simulink model "GFMUPS100k_CPP"  (R2024b)
settings: Solver=ode2  StartTime=0.0  StopTime=6  FixedStep=5e-7  RelTol=1e-3
model workspace (MAT data in the model file):
  amp = 0
  f1 = 1000
undefined symbols (not defined in the file or in its folder): DiscIntNeverNeededParam, L
libraries: spsIGBTDiodeLib x12, slpidlib x12, spsabctodq0Lib x10, spsSeriesRLCBranchLib x9, spsPLL3phLib x8, spsThreePhaseSeriesRLCBranchLib x8, spsDiodeLib x6, dspstat3 x5, spsVoltageMeasurementLib x4, spsThreePhaseVIMeasurementLib x4, spsPower3phInstantaneousLib x3, spsControlledCurrentSourceLib x3
(part 1 of 4)
settings Model: SimulationMode=accelerator  PacingRate=1000  Creator=Administrator  LastModifiedBy=zzc

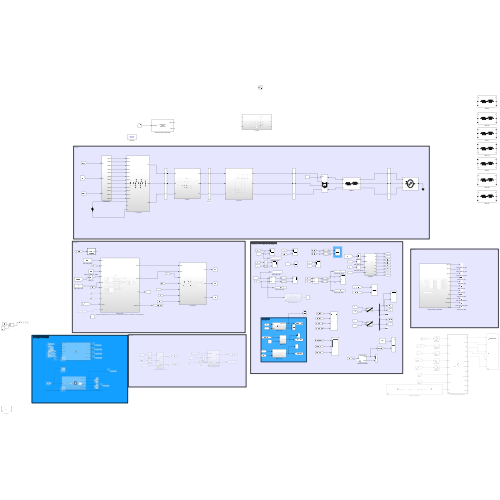
[thumbnail: Simulink's stored preview of the top-level diagram]
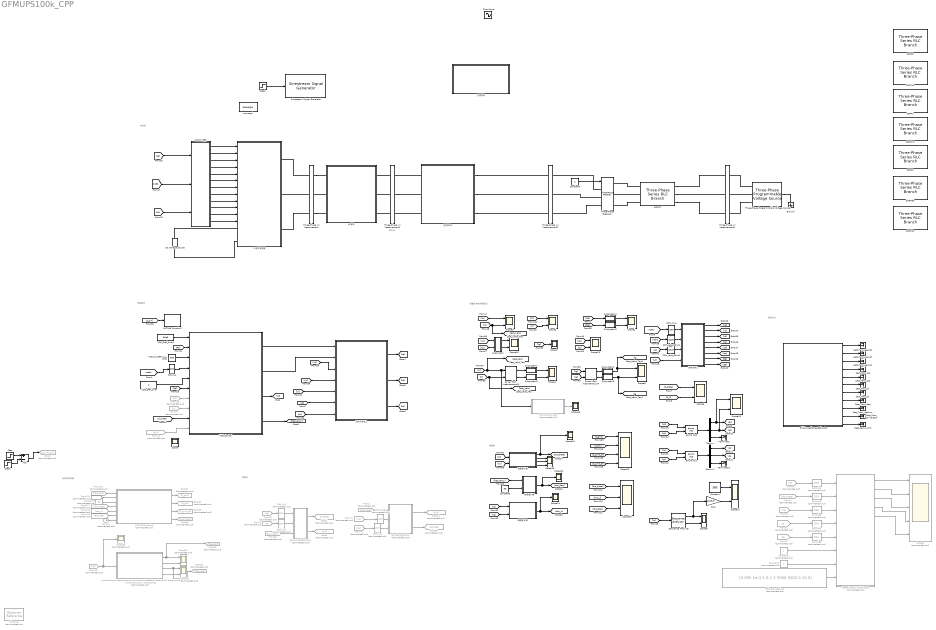
== system GFMUPS100k_CPP ==
  note: 阻抗估计
  note: PCC点
  note: 控制部分
  note: 主电路
  note: 相角差
  note: 测量与坐标转换部分
  note: 合闸信号判断
  note: 预同步
  A practical and fast sequence components detection scheme for three-phase unbalanced grid voltage.2021 : Subsystem  Commented=on
  Add : Sum  Inputs=+-
  Clock2 : Clock  Commented=on
  Constant : Constant  Value=380
  Constant1 : Constant  Commented=on
  Constant2 : Constant  Commented=on  Value=0
  Constant3 : Constant  Value=50
  Constant4 : Constant
  Constant5 : Constant  Commented=on  Value=50
  DC Voltage Source : spsDCVoltageSourceLib/DC Voltage Source  Amplitude=1500  Measurements=None
  Demux : Demux  Outputs=3
  Demux1 : Demux  Outputs=3
  Estimator_Settings : Constant  Commented=on  Value=[0.005 1e-4 5 0.1 5 5000 5000 0.15 0]
  From{10,40,74,121} (4 alike) : From  Commented=on  GotoTag=Vg  TagVisibility=global
  From11 : From  Commented=on  GotoTag=Qg  TagVisibility=global
  From116 : From  Commented=on  GotoTag=cha_freq
  From117 : From  Commented=on  GotoTag=cha_theta
  From118 : From  Commented=on  GotoTag=cha_U
  From119 : From  Commented=on  GotoTag=Mag_pos
  From12 : From  Commented=on  GotoTag=Pg  TagVisibility=global
  From120 : From  Commented=on  GotoTag=Mag_neg
  From2 : From  Commented=on  GotoTag=S_sync_en
  From26 : From  Commented=on  GotoTag=id
  From27 : From  Commented=on  GotoTag=iq
  From39 : From  Commented=on  GotoTag=S_sync_en
  From42 : From  Commented=on  GotoTag=Vs  TagVisibility=global
  From44 : From  Commented=on  GotoTag=d_U
  From73 : From  Commented=on  GotoTag=Vs  TagVisibility=global
  From8 : From  Commented=on  GotoTag=Vs  TagVisibility=global
  From9 : From  Commented=on  GotoTag=cha_theta
  Gain : Gain  Gain=sqrt(3/2)
  Goto39 : Goto  Commented=on  GotoTag=d_theta
  Goto40 : Goto  Commented=on  GotoTag=d_U
  Goto54 : Goto  Commented=on  GotoTag=Mag_pos
  Goto55 : Goto  Commented=on  GotoTag=Mag_neg
  Goto57 : Goto  Commented=on  GotoTag=S_grid
  Goto58 : Goto  Commented=on  GotoTag=S_sync_en
  Goto59 : Goto  Commented=on  GotoTag=S_sync_ok
  Goto60 : Goto  Commented=on  GotoTag=S_brk
  Goto7 : Goto  Commented=on  GotoTag=d_theta
  Goto8 : Goto  Commented=on  GotoTag=d_U
  Goto9 : Goto  Commented=on  GotoTag=S_sync_en
  Grid_Impedance_Estimator : Subsystem
  Ground : spsGroundLib/Ground  LConnTagsString=a
  IEC 62040-3-Test : Subsystem  Commented=on
  LC滤波 : Subsystem
  MATLAB Function2 : MATLAB Function  TreatAsAtomicUnit=on
  MATLAB Function3 : MATLAB Function  Commented=on  TreatAsAtomicUnit=on  SystemSampleTime=5e-05
  Observer : ObserverReference  Commented=on  ObserverModelName=GFMUPS100k_T1_Observer1
  Operating_Point_Estimator : MATLAB Function  Commented=on  TreatAsAtomicUnit=on
  "Power (3ph, Instantaneous)3" : spsPower3phInstantaneousLib/Power (3ph, Instantaneous)
  "Power (3ph, Instantaneous)4" : spsPower3phInstantaneousLib/Power (3ph, Instantaneous)
  SCR=1 : spsThreePhaseSeriesRLCBranchLib/Three-Phase Series RLC Branch  LConnTagsString=A|B|C  RConnTagsString=A|B|C  BranchType=RL  Resistance=0.1436835  Inductance=0.004573584  Capacitance=1e-6  Measurements=None
  SCR=1.5 : spsThreePhaseSeriesRLCBranchLib/Three-Phase Series RLC Branch  LConnTagsString=A|B|C  RConnTagsString=A|B|C  BranchType=RL  Resistance=0.095789  Inductance=0.003049056  Capacitance=1e-6  Measurements=None
  SCR=10 : spsThreePhaseSeriesRLCBranchLib/Three-Phase Series RLC Branch  LConnTagsString=A|B|C  RConnTagsString=A|B|C  BranchType=RL  Resistance=0.014368  Inductance=0.000457358  Capacitance=1e-6  Measurements=None
  SCR=2 : spsThreePhaseSeriesRLCBranchLib/Three-Phase Series RLC Branch  LConnTagsString=A|B|C  RConnTagsString=A|B|C  BranchType=RL  Resistance=0.047894  Inductance=0.001524528  Capacitance=1e-6  Measurements=None
  SCR=3 : spsThreePhaseSeriesRLCBranchLib/Three-Phase Series RLC Branch  LConnTagsString=A|B|C  RConnTagsString=A|B|C  BranchType=RL  Resistance=0.047894  Inductance=0.001524528  Capacitance=1e-6  Measurements=None
  SCR=30 : spsThreePhaseSeriesRLCBranchLib/Three-Phase Series RLC Branch  LConnTagsString=A|B|C  RConnTagsString=A|B|C  BranchType=RL  Resistance=0.004789  Inductance=0.000152453  Capacitance=1e-6  Measurements=None
  SCR=40 : spsThreePhaseSeriesRLCBranchLib/Three-Phase Series RLC Branch  LConnTagsString=A|B|C  RConnTagsString=A|B|C  BranchType=RL  Resistance=0.003592088  Inductance=0.0001143396  Capacitance=1e-6  Measurements=None
  SCR=5 : spsThreePhaseSeriesRLCBranchLib/Three-Phase Series RLC Branch  LConnTagsString=A|B|C  RConnTagsString=A|B|C  BranchType=RL  Resistance=0.028736674  Inductance=0.914716745e-3  Capacitance=1e-6  Measurements=None
  SVPWM调制 : Subsystem
  Sample{1..5} (5 alike) : ZeroOrderHold  Commented=on  SampleTime=1e-4
  Scope{,7,14,16,19..20} (6 alike) : Scope
  Scope{1..6,9..10,13,15,17} (11 alike) : Scope  NumInputPorts=2
  Scope11 : Scope  Commented=on  NumInputPorts=2
  Scope12 : Scope  Commented=on  NumInputPorts=2
  Scope18 : Scope  NumInputPorts=3
  Scope23 : Scope  Commented=on
  Scope24 : Scope  NumInputPorts=4
  Scope25 : Scope  NumInputPorts=3
  Scope8 : Scope  Commented=on  NumInputPorts=5
  Sequence Analyzer : eeSequenceAnalyzer/Sequence Analyzer  VariantControl=Variant1  LabelModeActiveChoice=Continuous  F=50  K=1  Seq=Positive  Ts=0
      settings: LibrarySourceBlock=ee_sl_lib/Measurements/Sequence Analyzer
  Sine Wave : Sin  SampleTime=0
  Sinestream Signal Generator : slctrl_signal/Sinestream Signal Generator  DiscreteTs=1e-4  BlockDataType=double  SignalSource=Block parameters  Frequencies=[20 40 60 100]  FreqUnits=Hz  Amplitudes=[1.07 1.07 1.07 1.07]  NumOfFreq=3  NumOfSignalPeriod=6  SinestreamType=sine  PhaseShift=0  PhaseShiftUnits=deg  ThreePhaseSignal=on  OutputFreqIndex=on  UseExternalTs=off  CompiledTsChoice=InternalTs  SinestreamSignalChoice=VariantSin3Phase
      settings: LibrarySourceBlock=slctrlblks/Signal Generation/Sinestream Signal Generator
  Step : Step  Time=0.3  SampleTime=0
  Step1 : Step  Time=0.85  SampleTime=0
  Step2 : Step  Time=0.5  SampleTime=0
  Subsystem : Subsystem
  Subsystem1 : Subsystem
  Subsystem2 : Subsystem
  Subsystem3 : Subsystem
  Subsystem4 : Subsystem
  Subsystem7 : Subsystem
  Subsystem8 : Subsystem
  Terminator : Terminator
  Terminator1 : Terminator
  Three-Phase Programmable Voltage Source : spsThreePhaseProgrammableVoltageSourceLib/Three-Phase Programmable Voltage Source  PositiveSequence="[380  0 50]"  VariationEntity=None  VariationType=Step  VariationTypeAlt=Step  VariationStep=-0.2  VariationRate=10  VariationMagnitude=0.3  VariationFrequency=2  VariationTiming=[1.5 2.4]  VariationPhaseA=off  Amplitudes=[1 0.8 1.2 1.0]  TimeValues=[0 0.1 0.15 0.2]  HarmonicGeneration=off  HarmonicA=[3 0.2 -25 0]  HarmonicB=[2 0.15 35 2]  Timing="[0.05  3]"  BusType=swing  Pref=0  Qref=0  Qmin=-inf  Qmax=inf
  Three-Phase V-I Measurement : spsThreePhaseVIMeasurementLib/Three-Phase V-I Measurement  VoltageMeasurement=no  SetLabelV=off  LabelV=Vabc  Vpu=off  VpuLL=off  CurrentMeasurement=yes  SetLabelI=on  LabelI=Iabc  Ipu=off  Pbase=100e6  Vbase=500e3  OutputType=Complex  PhasorSimulation=off  PSBequivalent=0
  Three-Phase V-I Measurement1 : spsThreePhaseVIMeasurementLib/Three-Phase V-I Measurement  VoltageMeasurement=phase-to-ground  SetLabelV=on  LabelV=Vs  Vpu=off  VpuLL=off  CurrentMeasurement=yes  SetLabelI=on  LabelI=Is  Ipu=off  Pbase=100e6  Vbase=500e3  OutputType=Complex  PhasorSimulation=off  PSBequivalent=0
  Three-Phase V-I Measurement2 : spsThreePhaseVIMeasurementLib/Three-Phase V-I Measurement  VoltageMeasurement=phase-to-ground  SetLabelV=on  LabelV=Vg  Vpu=off  VpuLL=off  CurrentMeasurement=yes  SetLabelI=on  LabelI=Ig  Ipu=off  Pbase=100e6  Vbase=500e3  OutputType=Complex  PhasorSimulation=off  PSBequivalent=0
  Three-Phase V-I Measurement4 : spsThreePhaseVIMeasurementLib/Three-Phase V-I Measurement  VoltageMeasurement=phase-to-ground  SetLabelV=on  LabelV=V1  Vpu=off  VpuLL=off  CurrentMeasurement=yes  SetLabelI=on  LabelI=I1  Ipu=off  Pbase=100e6  Vbase=500e3  OutputType=Complex  PhasorSimulation=off  PSBequivalent=0
  Three-Phase Breaker1 : spsThreePhaseBreakerLib/Three-Phase Breaker  InitialState=closed  SwitchA=on  SwitchB=on  SwitchC=on  SwitchTimes="[1  2]"  External=on  BreakerResistance=1e-6  SnubberResistance=1e6  SnubberCapacitance=inf  Measurements=None
  VSG_Control : Subsystem
      settings: AttributesFormatString=Reviewed discrete VSG, Ts=100 us; Q-U retuned to 0.5 Hz for real NPC; L1/R1 bypassed
  VSG_Qref_0var : Constant  Value=0  SampleTime=100e-6
  VSG_Qref_0var1 : Constant  Value=80e3  SampleTime=100e-6
  VSG_Un_380V_LL_RMS : Constant  Value=380  SampleTime=100e-6
  ZOH_Iabc_50us1 : ZeroOrderHold  SampleTime=50e-6
  ZOH_Iabc_50us2 : ZeroOrderHold  SampleTime=50e-6
  ZOH_Vs : ZeroOrderHold  SampleTime=5e-05
  ZOH_Vs{1..4} (4 alike) : ZeroOrderHold  Commented=on  SampleTime=5e-05
  ZOH_Vs_1 : ZeroOrderHold  SampleTime=5e-6
  Zest_Term_Lg_hat : Terminator
  Zest_Term_Pg : Terminator
  Zest_Term_Qg : Terminator
  Zest_Term_Rg_hat : Terminator
  Zest_Term_Xg_hat : Terminator
  Zest_Term_converged : Terminator
  Zest_Term_detJ : Terminator
  Zest_Term_f1 : Terminator
  Zest_Term_f2 : Terminator
  Zest_Term_iterNum : Terminator
  Zest_Term_valid : Terminator
  abc to dq0 : spsabctodq0Lib/abc to dq0  Alignment=90 degrees behind phase A axis
  abc to dq1 : spsabctodq0Lib/abc to dq0  Alignment=90 degrees behind phase A axis
  powergui : spspowerguiLib/powergui  Priority=1  SimulationMode=Discrete  SampleTime=5e-7  frequency=60  Iterations=50  frequencyindice=0  Pbase=100e6  ErrMax=1e-4  UnitsV=kV  UnitsW=MW  buscounter=0  FunctionMessages=off  echomessages=off  EnableUseOfTLC=off  CurrentSourceSwitches=off  DisableSnubberDevices=off  DisableRonSwitches=off  DisableVfSwitches=off  DisplayEquations=off  AutomaticDiscreteSolvers=off  SolverType=Tustin/Backward Euler (TBE)  Interpol=off  ExternalGateDelay=off  methode=off  Ts=100  x0status=blocks  SPID=on  SwTol=0  HookPort=off  NonlinearTolerance=1e-4  nMaxIteration=100  ContinueOnMaxIteration=off  RestoreLinks=warning  ResistiveCurrentMeasurement=off  Frange=[0:2:500]  Ylog=off  Xlog=on  ShowGrid=off  save=off  variable=ZData  structure=0  ZoomFFT=off  StartTime=0.0  cycles=1  DisplayStyle=1  fundamental=60  FreqAxis=off  MaxFrequency=1000  frequencyindicesteady=1  RmsSteady=1  display=off
  三电平逆变器 : Subsystem
  双闭环控制1 : Subsystem
  坐标变换1 : Subsystem
  基于自适应虚拟电流 : Subsystem  Commented=on
  基于转dq的预同步控制1 : Subsystem  Commented=on
  幅值差计算 : Subsystem
  正序扰动 : Subsystem
  正序扰动1 : Subsystem
  相角差计算 : Subsystem
  频率差计算 : Subsystem
  tag scope: Pg=global, Qg=global, Vgd=global, Vgq=global, Vsd=global, Vsq=global, Zest_ILabc=global, Zest_Iuabc=global, Zest_Vabc=global
  wires:
  SVPWM调制/1(PWM1) -> 三电平逆变器/1(pwm1)
  SVPWM调制/2(PWM2) -> 三电平逆变器/2(pwm2)
  SVPWM调制/3(PWM3) -> 三电平逆变器/3(pwm3)
  SVPWM调制/4(PWM4) -> 三电平逆变器/4(pwm4)
  SVPWM调制/5(PWM5) -> 三电平逆变器/5(pwm5)
  SVPWM调制/6(PWM6) -> 三电平逆变器/6(pwm6)
  SVPWM调制/7(PWM7) -> 三电平逆变器/7(pwm7)
  SVPWM调制/8(PWM8) -> 三电平逆变器/8(pwm8)
  SVPWM调制/9(PWM9) -> 三电平逆变器/9(pwm9)
  SVPWM调制/10(PWM10) -> 三电平逆变器/10(pwm10)
  SVPWM调制/11(PWM11) -> 三电平逆变器/11(pwm11)
  SVPWM调制/12(PWM12) -> 三电平逆变器/12(pwm12)
  VSG_Un_380V_LL_RMS/1 -> VSG_Control/3(Un)
  VSG_Qref_0var/1 -> VSG_Control/5(Qref)
  VSG_Control/3(wt) -> [wt]
  坐标变换1/2(vq) -> [vq]
  坐标变换1/5(isd) -> [isd]
  坐标变换1/1(vd) -> [vd]
  坐标变换1/7(Pe) -> [Pe]
  坐标变换1/8(Qe) -> [Qe]
  [wt] -> 坐标变换1/4(wt)
  坐标变换1/4(iq) -> [iq]
  [Iabc] -> ZOH_Iabc_50us1/1
  [Is] -> ZOH_Iabc_50us2/1
  坐标变换1/6(isq) -> [isq]
  坐标变换1/3(id) -> [id]
  [Vcabc] -> ZOH_Vs_1/1
  ZOH_Vs_1/1 -> 坐标变换1/1(Vs)
  ZOH_Iabc_50us1/1 -> 坐标变换1/2(Iabc)
  ZOH_Iabc_50us2/1 -> 坐标变换1/3(Is)
  [Ua] -> SVPWM调制/1(ua)
  [Ub] -> SVPWM调制/2(ub)
  [Uc] -> SVPWM调制/3(uc)
  [Pe] -> VSG_Control/2(Pe)
  [Qe] -> VSG_Control/6(Qe)
  From26/1 -> VSG_Control/7(id)
  From27/1 -> VSG_Control/8(iq)
  [Vcabc] -> ZOH_Vs/1
  ZOH_Vs/1 -> VSG_Control/4(Vs)
  VSG_Control/4(frequency) -> [frequency]
  [iq] -> 双闭环控制1/6(iq)
  双闭环控制1/3(UC) -> [Uc]
  [id] -> 双闭环控制1/5(id)
  双闭环控制1/2(UB) -> [Ub]
  [vd] -> 双闭环控制1/3(Vd)
  双闭环控制1/1(UA) -> [Ua]
  [wt] -> 双闭环控制1/7(wt)
  [vq] -> 双闭环控制1/4(Vq)
  From40/1 -> ZOH_Vs1/1
  基于转dq的预同步控制1/1(c_theta) -> Goto7/1
  From42/1 -> ZOH_Vs2/1
  基于转dq的预同步控制1/2(d_U) -> Goto8/1
  From39/1 -> 基于转dq的预同步控制1/3(presignal)
  [d_theta] -> VSG_Control/9(d_theta)
  From44/1 -> VSG_Control/10(d_U)
  Add/1 -> Goto9/1
  Step/1 -> Add/1
  Step1/1 -> Add/2
  [S_sync_ok] -> Scope24/3
  "Power (3ph, Instantaneous)4"/1 -> Subsystem1/1(In1)
  [cha_freq] -> Scope25/3
  [V1] -> 相角差计算/2(abc1)
  [Vl] -> Scope2/1
  相角差计算/3(Out3) -> Scope18/2
  [Vl] -> IEC 62040-3-Test/1(In1), "Power (3ph, Instantaneous)3"/1, [Zest_Vabc]
  Subsystem/2(Out2) -> Scope10/2
  Subsystem/1(Out1) -> Scope10/1
  [Vs] -> Subsystem/1(In1)
  "Power (3ph, Instantaneous)3"/2 -> Subsystem8/1(In1)
  "Power (3ph, Instantaneous)4"/2 -> Subsystem2/1(In1)
  "Power (3ph, Instantaneous)3"/1 -> Subsystem7/1(In1)
  [Ig] -> "Power (3ph, Instantaneous)4"/2
  [Vg] -> Scope13/1
  [frequency] -> 频率差计算/1(In1)
  [Vg] -> Subsystem/2(In2)
  频率差计算/1(Out1) -> Scope20/1, [cha_freq]
  [Vs] -> 相角差计算/1(abc)
  相角差计算/1(dete_theta) -> Scope19/1, [cha_theta]
  [S_grid] -> Scope24/1
  相角差计算/4(Out4) -> Scope18/3
  [Vs] -> Scope3/1  "Vs"
  [Vg] -> 幅值差计算/2(In2)
  [S_sync_en] -> Scope24/4
  IEC 62040-3-Test/1(Out1) -> Scope16/1
  [Il] -> Scope2/2
  幅值差计算/1(Out1) -> Scope14/1, [cha_U]
  [Vg] -> Scope7/1
  [Il] -> "Power (3ph, Instantaneous)3"/2, [Zest_ILabc]
  [cha_theta] -> Scope25/1
  Constant3/1 -> 频率差计算/2(In2)
  相角差计算/2(Out2) -> Scope18/1
  [Ig] -> Scope13/2
  [Vg] -> "Power (3ph, Instantaneous)4"/1
  [S_brk] -> Scope24/2
  [Vs] -> 幅值差计算/1(In1)
  [cha_U] -> Scope25/2
  Subsystem1/1(Out1) -> [Pg], Scope5/1  "Pg"
  Subsystem2/1(Out1) -> [Qg], Scope5/2  "Qg"
  Subsystem7/1(Out1) -> Scope4/1
  Subsystem8/1(Out1) -> Scope4/2
  [Pe] -> Subsystem4/1(In1)  "Pe"
  [Qe] -> Subsystem3/1(In1)  "Qe"
  ZOH_Vs1/1 -> 基于转dq的预同步控制1/1(Vg)
  ZOH_Vs2/1 -> 基于转dq的预同步控制1/2(Vabc)
  [Is] -> Scope3/2, [Zest_Iuabc]  "Is"
  VSG_Control/1(Vdref) -> 双闭环控制1/1(Vdref)
  VSG_Control/2(Vqref) -> 双闭环控制1/2(Vqref)
  MATLAB Function3/4(S_sync_en) -> Goto58/1
  From120/1 -> MATLAB Function3/2(v2_pu)
  A practical and fast sequence components detection scheme for three-phase unbalanced grid voltage.2021/4(Angle_neg) -> Scope12/2
  MATLAB Function3/2(S_brk) -> Goto60/1
  Constant5/1 -> MATLAB Function3/3(freq_hz)
  Clock2/1 -> MATLAB Function3/7(t)
  From116/1 -> MATLAB Function3/6(d_f)
  MATLAB Function3/1(S_grid) -> Goto57/1
  A practical and fast sequence components detection scheme for three-phase unbalanced grid voltage.2021/2(Angle_pos) -> Scope11/2
  From121/1 -> Scope23/1, A practical and fast sequence components detection scheme for three-phase unbalanced grid voltage.2021/1(In1)
  A practical and fast sequence components detection scheme for three-phase unbalanced grid voltage.2021/3(Mag_neg) -> Scope12/1, Goto55/1
  A practical and fast sequence components detection scheme for three-phase unbalanced grid voltage.2021/1(Mag_pos) -> Scope11/1, Goto54/1
  From117/1 -> MATLAB Function3/4(d_theta)
  From118/1 -> MATLAB Function3/5(d_U)
  From119/1 -> MATLAB Function3/1(v1_pu)
  MATLAB Function3/3(S_sync_ok) -> Goto59/1
  From2/1 -> 基于自适应虚拟电流/1(presignal)
  From74/1 -> ZOH_Vs4/1
  基于自适应虚拟电流/2(deta_w) -> Goto39/1
  基于自适应虚拟电流/1(deta_U) -> Goto40/1
  From73/1 -> ZOH_Vs3/1
  [d_theta] -> Scope6/1
  [d_U] -> Scope6/2
  ZOH_Vs3/1 -> 基于自适应虚拟电流/2(Vs_abc)
  ZOH_Vs4/1 -> 基于自适应虚拟电流/3(Vg_abc1)
  [S_brk] -> MATLAB Function2/1(S_brk)
  Step2/1 -> Sinestream Signal Generator/1
  Grid_Impedance_Estimator/1(Rg_hat) -> Zest_Term_Rg_hat/1
  Grid_Impedance_Estimator/2(Xg_hat) -> Zest_Term_Xg_hat/1
  Grid_Impedance_Estimator/3(Lg_hat) -> Zest_Term_Lg_hat/1
  Grid_Impedance_Estimator/4(Pg) -> Zest_Term_Pg/1
  Grid_Impedance_Estimator/5(Qg) -> Zest_Term_Qg/1
  Grid_Impedance_Estimator/6(f1) -> Zest_Term_f1/1
  Grid_Impedance_Estimator/7(f2) -> Zest_Term_f2/1
  Grid_Impedance_Estimator/8(detJ) -> Zest_Term_detJ/1
  Grid_Impedance_Estimator/9(iterNum) -> Zest_Term_iterNum/1
  Grid_Impedance_Estimator/10(converged) -> Zest_Term_converged/1
  Grid_Impedance_Estimator/11(valid) -> Zest_Term_valid/1
  From8/1 -> Sample1/1  "Vs"
  From9/1 -> Sample2/1
  From10/1 -> Sample3/1
  From11/1 -> Sample5/1
  From12/1 -> Sample4/1
  Constant2/1 -> Operating_Point_Estimator/7(reset)
  Sample1/1 -> Operating_Point_Estimator/1(E)
  Sample2/1 -> Operating_Point_Estimator/2(theta)
  Sample3/1 -> Operating_Point_Estimator/3(Vg)
  Sample4/1 -> Operating_Point_Estimator/4(Pg)
  Sample5/1 -> Operating_Point_Estimator/5(Qg)
  Constant1/1 -> Operating_Point_Estimator/6(enable)
  Estimator_Settings/1 -> Operating_Point_Estimator/8(cfg)
  Operating_Point_Estimator/1(E0) -> Scope8/1
  Operating_Point_Estimator/2(theta0) -> Scope8/2
  Operating_Point_Estimator/3(Vg0) -> Scope8/3
  Operating_Point_Estimator/4(Pg0) -> Scope8/4
  Operating_Point_Estimator/5(Qg0) -> Scope8/5
  Constant4/1 -> Three-Phase Breaker1/1
  [V1] -> abc to dq0/1
  [wt] -> abc to dq0/2
  Demux/2 -> Scope15/2, [Vgq]
  abc to dq0/1 -> Demux/1
  Demux/3 -> Terminator/1
  Demux/1 -> Scope15/1, [Vgd]
  Demux1/3 -> Terminator1/1
  abc to dq1/1 -> Demux1/1
  Demux1/2 -> [Vsq]
  [wt] -> abc to dq1/2
  [Vs] -> abc to dq1/1
  Demux1/1 -> [Vsd]
  Constant/1 -> Scope17/1
  Gain/1 -> Scope17/2
  Sequence Analyzer/2 -> Scope9/2
  [Vs] -> Sequence Analyzer/1  "Vs"
  Sequence Analyzer/1 -> Gain/1, Scope9/1
  VSG_Qref_0var1/1 -> VSG_Control/1(Pref)
  Subsystem4/1(Out1) -> Scope1/1  "Pg"
  Subsystem3/1(Out1) -> Scope1/2  "Qg"
  connections:
  DC Voltage Source/RConn1 -- 三电平逆变器/LConn1
  DC Voltage Source/LConn1 -- 三电平逆变器/LConn3
  Three-Phase V-I Measurement/LConn1 -- 三电平逆变器/RConn1
  Three-Phase V-I Measurement/LConn2 -- 三电平逆变器/RConn2
  Three-Phase V-I Measurement/LConn3 -- 三电平逆变器/RConn3
  LC滤波/LConn2 -- Three-Phase V-I Measurement/RConn2
  Three-Phase V-I Measurement/RConn1 -- LC滤波/LConn1
  Three-Phase V-I Measurement/RConn3 -- LC滤波/LConn3
  Three-Phase V-I Measurement1/LConn1 -- LC滤波/RConn1
  Three-Phase V-I Measurement1/LConn2 -- LC滤波/RConn2
  Three-Phase V-I Measurement1/LConn3 -- LC滤波/RConn3
  Three-Phase Breaker1/LConn2 -- Three-Phase V-I Measurement2/RConn2
  Three-Phase Breaker1/LConn3 -- Three-Phase V-I Measurement2/RConn3
  SCR=2/RConn2 -- Three-Phase V-I Measurement4/LConn2
  Three-Phase Breaker1/LConn1 -- Three-Phase V-I Measurement2/RConn1
  Three-Phase Programmable Voltage Source/LConn1 -- Ground/LConn1
  正序扰动1/RConn3 -- Three-Phase V-I Measurement2/LConn3
  正序扰动1/LConn1 -- Three-Phase V-I Measurement1/RConn1
  Three-Phase V-I Measurement1/RConn2 -- 正序扰动1/LConn2
  正序扰动1/LConn3 -- Three-Phase V-I Measurement1/RConn3
  SCR=2/LConn1 -- Three-Phase Breaker1/RConn1
  SCR=2/LConn2 -- Three-Phase Breaker1/RConn2
  SCR=2/LConn3 -- Three-Phase Breaker1/RConn3
  Three-Phase Programmable Voltage Source/RConn1 -- Three-Phase V-I Measurement4/RConn1
  Three-Phase Programmable Voltage Source/RConn2 -- Three-Phase V-I Measurement4/RConn2
  Three-Phase Programmable Voltage Source/RConn3 -- Three-Phase V-I Measurement4/RConn3
  SCR=2/RConn3 -- Three-Phase V-I Measurement4/LConn3
  SCR=2/RConn1 -- Three-Phase V-I Measurement4/LConn1
  正序扰动1/RConn1 -- Three-Phase V-I Measurement2/LConn1
  正序扰动1/RConn2 -- Three-Phase V-I Measurement2/LConn2

== system GFMUPS100k_CPP/A practical and fast sequence components detection scheme for three-phase unbalanced grid voltage.2021 ==
  note: 滤波
  In1 : Inport
  MATLAB Function1 : MATLAB Function  TreatAsAtomicUnit=on
  Mux : Mux  Inputs=3
  PLL (3ph) : spsPLL3phLib/PLL (3ph)  Fmin=45  Par_Init=[0, 60]  ParK=[180, 3200, 1]  TcD=1e-4  MaxRateChangeFreq=12  FilterCutOffFreq=25  Ts=0  AGC=on
  Subsystem : Subsystem
  Subsystem1 : Subsystem
  T1\T2矩阵变换 : MATLAB Function  TreatAsAtomicUnit=on
  Terminator : Terminator
  Ubeta计算 : Subsystem
  标幺化1 : Subsystem
  Mag_pos : Outport
  Angle_pos : Outport  Port=2
  Mag_neg : Outport  Port=3
  Angle_neg : Outport  Port=4
  wires:
  Mux/1 -> T1\T2矩阵变换/2(U_beta)
  Ubeta计算/1(uA_beta) -> Mux/1
  Ubeta计算/3(uC_beta) -> Mux/3
  标幺化1/1(U_alpha) -> Ubeta计算/1(In1), T1\T2矩阵变换/1(U_alpha)
  Ubeta计算/2(uB_beta) -> Mux/2
  In1/1 -> 标幺化1/1(In1)
  T1\T2矩阵变换/1(U_pos) -> PLL (3ph)/1, Subsystem/1(abc)
  PLL (3ph)/1 -> Terminator/1
  MATLAB Function1/1(Mag_pos) -> Mag_pos/1
  MATLAB Function1/2(Angle_pos) -> Angle_pos/1
  MATLAB Function1/3(Mag_neg) -> Mag_neg/1
  MATLAB Function1/4(Angle_neg) -> Angle_neg/1
  Subsystem1/2(uq_fliter) -> MATLAB Function1/4(Uq_neg)
  T1\T2矩阵变换/2(U_neg) -> Subsystem1/1(abc)
  Subsystem1/1(ud_fliter) -> MATLAB Function1/3(Ud_neg)
  Subsystem/2(uq_fliter) -> MATLAB Function1/2(Uq_pos)
  PLL (3ph)/2 -> Subsystem1/2(In1), MATLAB Function1/5(wt)
  Subsystem/1(ud_fliter) -> MATLAB Function1/1(Ud_pos)

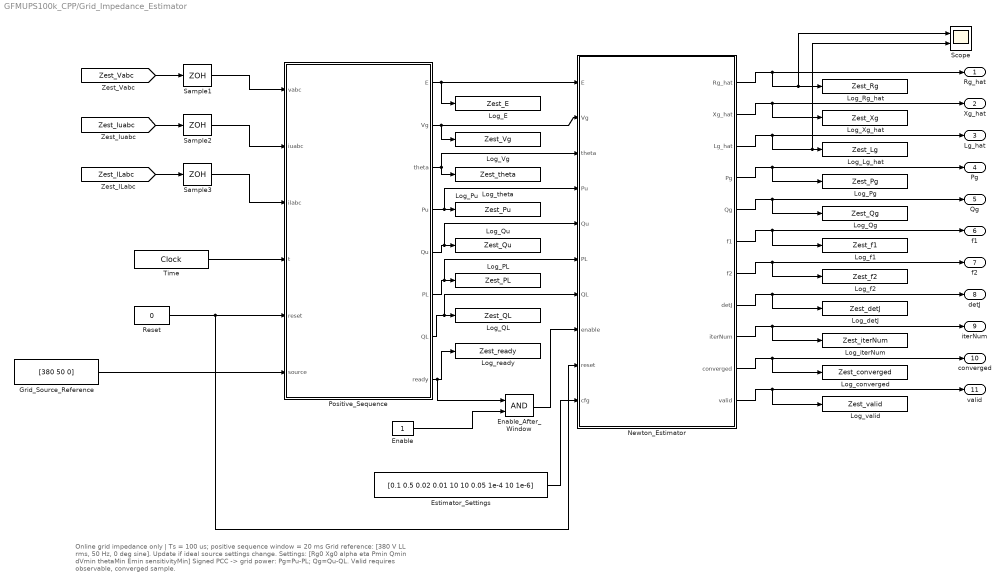
== system GFMUPS100k_CPP/Grid_Impedance_Estimator ==
  note: Online grid impedance only | Ts = 100 us; positive sequence window = 20 ms
      | Grid reference: [380 V LL rms, 50 Hz, 0 deg sine]. Update if ideal source settings change.
      | Settings: [Rg0 Xg0 alpha eta Pmin Qmin dVmin thetaMin Emin sensitivityMin]
      | Signed PCC -> grid power: Pg=Pu-PL; Qg=Qu-QL. Valid requires observable, converged sample.
  Enable : Constant  OutDataTypeStr=boolean
  Enable_After_Window : Logic
  Estimator_Settings : Constant  Value=[0.1 0.5 0.02 0.01 10 10 0.05 1e-4 10 1e-6]
  Grid_Source_Reference : Constant  Value=[380 50 0]
  Log_E : ToWorkspace  VariableName=Zest_E  SaveFormat=Timeseries  SampleTime=-1
  Log_Lg_hat : ToWorkspace  VariableName=Zest_Lg  SaveFormat=Timeseries  SampleTime=-1
  Log_PL : ToWorkspace  VariableName=Zest_PL  SaveFormat=Timeseries  SampleTime=-1
  Log_Pg : ToWorkspace  VariableName=Zest_Pg  SaveFormat=Timeseries  SampleTime=-1
  Log_Pu : ToWorkspace  VariableName=Zest_Pu  SaveFormat=Timeseries  SampleTime=-1
  Log_QL : ToWorkspace  VariableName=Zest_QL  SaveFormat=Timeseries  SampleTime=-1
  Log_Qg : ToWorkspace  VariableName=Zest_Qg  SaveFormat=Timeseries  SampleTime=-1
  Log_Qu : ToWorkspace  VariableName=Zest_Qu  SaveFormat=Timeseries  SampleTime=-1
  Log_Rg_hat : ToWorkspace  VariableName=Zest_Rg  SaveFormat=Timeseries  SampleTime=-1
  Log_Vg : ToWorkspace  VariableName=Zest_Vg  SaveFormat=Timeseries  SampleTime=-1
  Log_Xg_hat : ToWorkspace  VariableName=Zest_Xg  SaveFormat=Timeseries  SampleTime=-1
  Log_converged : ToWorkspace  VariableName=Zest_converged  SaveFormat=Timeseries  SampleTime=-1
  Log_detJ : ToWorkspace  VariableName=Zest_detJ  SaveFormat=Timeseries  SampleTime=-1
  Log_f1 : ToWorkspace  VariableName=Zest_f1  SaveFormat=Timeseries  SampleTime=-1
  Log_f2 : ToWorkspace  VariableName=Zest_f2  SaveFormat=Timeseries  SampleTime=-1
  Log_iterNum : ToWorkspace  VariableName=Zest_iterNum  SaveFormat=Timeseries  SampleTime=-1
  Log_ready : ToWorkspace  VariableName=Zest_ready  SaveFormat=Timeseries  SampleTime=-1
  Log_theta : ToWorkspace  VariableName=Zest_theta  SaveFormat=Timeseries  SampleTime=-1
  Log_valid : ToWorkspace  VariableName=Zest_valid  SaveFormat=Timeseries  SampleTime=-1
  Newton_Estimator : MATLAB Function  TreatAsAtomicUnit=on
  Positive_Sequence : MATLAB Function  TreatAsAtomicUnit=on
  Reset : Constant  Value=0
  Sample1 : ZeroOrderHold  SampleTime=1e-4
  Sample2 : ZeroOrderHold  SampleTime=1e-4
  Sample3 : ZeroOrderHold  SampleTime=1e-4
  Scope : Scope  NumInputPorts=2
  Time : DigitalClock  SampleTime=1e-4
  Rg_hat : Outport
  Xg_hat : Outport  Port=2
  Lg_hat : Outport  Port=3
  Pg : Outport  Port=4
  Qg : Outport  Port=5
  f1 : Outport  Port=6
  f2 : Outport  Port=7
  detJ : Outport  Port=8
  iterNum : Outport  Port=9
  converged : Outport  Port=10
  valid : Outport  Port=11
  wires:
  [Zest_Vabc] -> Sample1/1
  [Zest_Iuabc] -> Sample2/1
  [Zest_ILabc] -> Sample3/1
  Sample1/1 -> Positive_Sequence/1(vabc)
  Sample2/1 -> Positive_Sequence/2(iuabc)
  Sample3/1 -> Positive_Sequence/3(ilabc)
  Time/1 -> Positive_Sequence/4(t)
  Reset/1 -> Positive_Sequence/5(reset), Newton_Estimator/9(reset)
  Grid_Source_Reference/1 -> Positive_Sequence/6(source)
  Positive_Sequence/1(E) -> Log_E/1, Newton_Estimator/1(E)
  Positive_Sequence/2(Vg) -> Newton_Estimator/2(Vg), Log_Vg/1
  Positive_Sequence/3(theta) -> Newton_Estimator/3(theta), Log_theta/1
  Positive_Sequence/4(Pu) -> Newton_Estimator/4(Pu), Log_Pu/1
  Positive_Sequence/5(Qu) -> Newton_Estimator/5(Qu), Log_Qu/1
  Positive_Sequence/6(PL) -> Newton_Estimator/6(PL), Log_PL/1
  Positive_Sequence/7(QL) -> Newton_Estimator/7(QL), Log_QL/1
  Positive_Sequence/8(ready) -> Log_ready/1, Enable_After_Window/1
  Enable/1 -> Enable_After_Window/2
  Enable_After_Window/1 -> Newton_Estimator/8(enable)
  Estimator_Settings/1 -> Newton_Estimator/10(cfg)
  Newton_Estimator/1(Rg_hat) -> Rg_hat/1, Scope/1, Log_Rg_hat/1
  Newton_Estimator/2(Xg_hat) -> Xg_hat/1, Log_Xg_hat/1
  Newton_Estimator/3(Lg_hat) -> Lg_hat/1, Scope/2, Log_Lg_hat/1
  Newton_Estimator/4(Pg) -> Pg/1, Log_Pg/1
  Newton_Estimator/5(Qg) -> Qg/1, Log_Qg/1
  Newton_Estimator/6(f1) -> f1/1, Log_f1/1
  Newton_Estimator/7(f2) -> f2/1, Log_f2/1
  Newton_Estimator/8(detJ) -> detJ/1, Log_detJ/1
  Newton_Estimator/9(iterNum) -> iterNum/1, Log_iterNum/1
  Newton_Estimator/10(converged) -> converged/1, Log_converged/1
  Newton_Estimator/11(valid) -> valid/1, Log_valid/1

== system GFMUPS100k_CPP/IEC 62040-3-Test ==
  In1 : Inport
  Add1 : Sum
  Demux : Demux  Outputs=3
  Gain : Gain  Gain=1/563
  PLL (3ph) : spsPLL3phLib/PLL (3ph)  Fmin=45  Par_Init=[0, 60]  ParK=[180, 3200, 1]  TcD=1e-4  MaxRateChangeFreq=12  FilterCutOffFreq=25  Ts=0  AGC=on
  Scope : Scope
  Sqrt : Sqrt
  Terminator : Terminator
  Terminator1 : Terminator
  abc to dq0 : spsabctodq0Lib/abc to dq0  Alignment=90 degrees behind phase A axis
  Out1 : Outport
  wires:
  Gain/1 -> abc to dq0/1, Scope/1
  Add1/1 -> Sqrt/1
  Demux/2 -> Add1/2
  In1/1 -> PLL (3ph)/1, Gain/1
  Demux/1 -> Add1/1
  Demux/3 -> Terminator/1
  abc to dq0/1 -> Demux/1
  Sqrt/1 -> Out1/1
  PLL (3ph)/2 -> abc to dq0/2
  PLL (3ph)/1 -> Terminator1/1

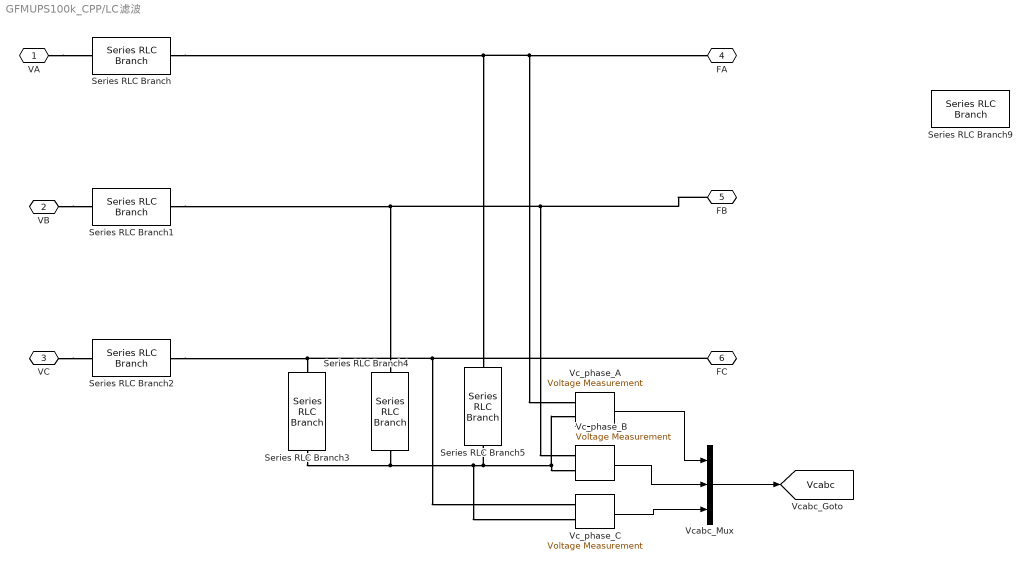
== system GFMUPS100k_CPP/LC滤波 ==
  Series RLC Branch : spsSeriesRLCBranchLib/Series RLC Branch  LConnTagsString=__new0  RConnTagsString=__new0  BranchType=RL  Resistance=0.01  Inductance=182e-6  SetiL0=off  InitialCurrent=0  Capacitance=1e-6  Setx0=off  InitialVoltage=0  Measurements=None
  Series RLC Branch1 : spsSeriesRLCBranchLib/Series RLC Branch  LConnTagsString=__new0  RConnTagsString=__new0  BranchType=RL  Resistance=0.01  Inductance=182e-6  SetiL0=off  InitialCurrent=0  Capacitance=1e-6  Setx0=off  InitialVoltage=0  Measurements=None
  Series RLC Branch2 : spsSeriesRLCBranchLib/Series RLC Branch  LConnTagsString=__new0  RConnTagsString=__new0  BranchType=RL  Resistance=0.01  Inductance=182e-6  SetiL0=off  InitialCurrent=0  Capacitance=1e-6  Setx0=off  InitialVoltage=0  Measurements=None
  Series RLC Branch3 : spsSeriesRLCBranchLib/Series RLC Branch  LConnTagsString=__new0  RConnTagsString=__new0  BranchType=RC  Resistance=0.01  Inductance=L  SetiL0=off  InitialCurrent=0  Capacitance=2.8e-05  Setx0=off  InitialVoltage=0  Measurements=None
  Series RLC Branch4 : spsSeriesRLCBranchLib/Series RLC Branch  LConnTagsString=__new0  RConnTagsString=__new0  BranchType=RC  Resistance=0.01  Inductance=L  SetiL0=off  InitialCurrent=0  Capacitance=2.8e-05  Setx0=off  InitialVoltage=0  Measurements=None
  Series RLC Branch5 : spsSeriesRLCBranchLib/Series RLC Branch  LConnTagsString=__new0  RConnTagsString=__new0  BranchType=RC  Resistance=0.01  Inductance=L  SetiL0=off  InitialCurrent=0  Capacitance=2.8e-05  Setx0=off  InitialVoltage=0  Measurements=None
  Series RLC Branch9 : spsSeriesRLCBranchLib/Series RLC Branch  LConnTagsString=__new0  RConnTagsString=__new0  BranchType=RL  Resistance=0.01  Inductance=5e-6  SetiL0=off  InitialCurrent=0  Capacitance=1e-6  Setx0=off  InitialVoltage=0  Measurements=None
  Vc_phase_A : spsVoltageMeasurementLib/Voltage Measurement  PhasorSimulation=off  OutputType=Complex  PSBequivalent=0
  Vc_phase_B : spsVoltageMeasurementLib/Voltage Measurement  PhasorSimulation=off  OutputType=Complex  PSBequivalent=0
  Vc_phase_C : spsVoltageMeasurementLib/Voltage Measurement  PhasorSimulation=off  OutputType=Complex  PSBequivalent=0
  Vcabc_Mux : Mux  Inputs=3
  VA : PMIOPort  Side=Left
  VB : PMIOPort  Port=2  Side=Left
  VC : PMIOPort  Port=3  Side=Left
  FA : PMIOPort  Port=4  Side=Right
  FB : PMIOPort  Port=5  Side=Right
  FC : PMIOPort  Port=6  Side=Right
  tag scope: Vcabc=global
  wires:
  Vcabc_Mux/1 -> [Vcabc]
  Vc_phase_A/1 -> Vcabc_Mux/1
  Vc_phase_B/1 -> Vcabc_Mux/2
  Vc_phase_C/1 -> Vcabc_Mux/3
  connections:
  FA/RConn1 -- Vc_phase_A/LConn1 -- Series RLC Branch/RConn1 -- Series RLC Branch5/LConn1
  VC/RConn1 -- Series RLC Branch2/LConn1
  VA/RConn1 -- Series RLC Branch/LConn1
  Series RLC Branch3/RConn1 -- Series RLC Branch4/RConn1 -- Series RLC Branch5/RConn1 -- Vc_phase_B/LConn2 -- Vc_phase_A/LConn2 -- Vc_phase_C/LConn2
  Series RLC Branch1/RConn1 -- FB/RConn1 -- Vc_phase_B/LConn1 -- Series RLC Branch4/LConn1
  VB/RConn1 -- Series RLC Branch1/LConn1
  FC/RConn1 -- Vc_phase_C/LConn1 -- Series RLC Branch2/RConn1 -- Series RLC Branch3/LConn1

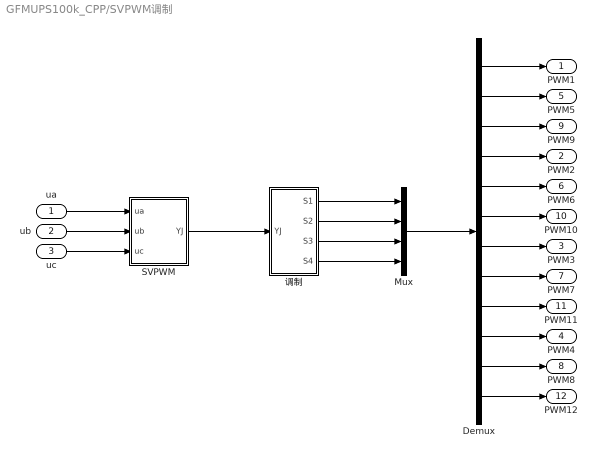
== system GFMUPS100k_CPP/SVPWM调制 ==
  ua : Inport
  ub : Inport  Port=2
  uc : Inport  Port=3
  Demux : Demux  Outputs=12
  Mux : Mux
  SVPWM : Subsystem
  调制 : Subsystem
  PWM1 : Outport
  PWM2 : Outport  Port=2
  PWM3 : Outport  Port=3
  PWM4 : Outport  Port=4
  PWM5 : Outport  Port=5
  PWM6 : Outport  Port=6
  PWM7 : Outport  Port=7
  PWM8 : Outport  Port=8
  PWM9 : Outport  Port=9
  PWM10 : Outport  Port=10
  PWM11 : Outport  Port=11
  PWM12 : Outport  Port=12
  wires:
  Demux/4 -> PWM2/1
  Demux/7 -> PWM3/1
  SVPWM/1(YJ) -> 调制/1(YJ)
  uc/1 -> SVPWM/3(uc)
  Mux/1 -> Demux/1
  Demux/1 -> PWM1/1
  Demux/12 -> PWM12/1
  ua/1 -> SVPWM/1(ua)
  Demux/11 -> PWM8/1
  Demux/10 -> PWM4/1
  Demux/2 -> PWM5/1
  Demux/9 -> PWM11/1
  Demux/5 -> PWM6/1
  ub/1 -> SVPWM/2(ub)
  Demux/6 -> PWM10/1
  Demux/8 -> PWM7/1
  Demux/3 -> PWM9/1
  调制/1(S1) -> Mux/1
  调制/2(S2) -> Mux/2
  调制/3(S3) -> Mux/3
  调制/4(S4) -> Mux/4

== system GFMUPS100k_CPP/Subsystem ==
  In1 : Inport
  In2 : Inport  Port=2
  Demux1 : Demux  Outputs=3
  Demux2 : Demux  Outputs=3
  Terminator{2..5} (4 alike) : Terminator
  Out1 : Outport
  Out2 : Outport  Port=2
  wires:
  Demux1/2 -> Terminator2/1
  Demux2/3 -> Terminator5/1
  Demux2/2 -> Terminator4/1
  In1/1 -> Demux1/1
  Demux1/3 -> Terminator3/1
  Demux2/1 -> Out2/1
  In2/1 -> Demux2/1
  Demux1/1 -> Out1/1

== system GFMUPS100k_CPP/Subsystem1 ==
  In1 : Inport
  Discrete-Time Integrator : DiscreteIntegrator  SampleTime=1/20000  ICPrevOutput=DiscIntNeverNeededParam  ICPrevScaledInput=DiscIntNeverNeededParam
  Gain1 : Gain  Gain=2*pi*50
  Gain2 : Gain
  Sum3 : Sum  Inputs=|+-
  Out1 : Outport
  wires:
  Sum3/1 -> Gain1/1
  Gain1/1 -> Discrete-Time Integrator/1
  Gain2/1 -> Sum3/2
  In1/1 -> Sum3/1
  Discrete-Time Integrator/1 -> Gain2/1, Out1/1

== system GFMUPS100k_CPP/Subsystem2 ==
  In1 : Inport
  Discrete-Time Integrator : DiscreteIntegrator  SampleTime=1/20000  ICPrevOutput=DiscIntNeverNeededParam  ICPrevScaledInput=DiscIntNeverNeededParam
  Gain1 : Gain  Gain=2*pi*50
  Gain2 : Gain
  Sum3 : Sum  Inputs=|+-
  Out1 : Outport
  wires:
  Discrete-Time Integrator/1 -> Out1/1, Gain2/1
  In1/1 -> Sum3/1
  Gain2/1 -> Sum3/2
  Gain1/1 -> Discrete-Time Integrator/1
  Sum3/1 -> Gain1/1

== system GFMUPS100k_CPP/Subsystem3 ==
  In1 : Inport
  Discrete-Time Integrator : DiscreteIntegrator  SampleTime=1/20000  ICPrevOutput=DiscIntNeverNeededParam  ICPrevScaledInput=DiscIntNeverNeededParam
  Gain1 : Gain  Gain=2*pi*10
  Gain2 : Gain
  Sum3 : Sum  Inputs=|+-
  Out1 : Outport
  wires:
  Sum3/1 -> Gain1/1
  Gain1/1 -> Discrete-Time Integrator/1
  Gain2/1 -> Sum3/2
  In1/1 -> Sum3/1
  Discrete-Time Integrator/1 -> Gain2/1, Out1/1

== system GFMUPS100k_CPP/Subsystem4 ==
  In1 : Inport
  Discrete-Time Integrator : DiscreteIntegrator  SampleTime=1/20000  ICPrevOutput=DiscIntNeverNeededParam  ICPrevScaledInput=DiscIntNeverNeededParam
  Gain1 : Gain  Gain=2*pi*10
  Gain2 : Gain
  Sum3 : Sum  Inputs=|+-
  Out1 : Outport
  wires:
  Sum3/1 -> Gain1/1
  Gain1/1 -> Discrete-Time Integrator/1
  Gain2/1 -> Sum3/2
  In1/1 -> Sum3/1
  Discrete-Time Integrator/1 -> Gain2/1, Out1/1

== system GFMUPS100k_CPP/Subsystem7 ==
  In1 : Inport
  Discrete-Time Integrator : DiscreteIntegrator  SampleTime=1/20000  ICPrevOutput=DiscIntNeverNeededParam  ICPrevScaledInput=DiscIntNeverNeededParam
  Gain1 : Gain  Gain=2*pi*50
  Gain2 : Gain
  Sum3 : Sum  Inputs=|+-
  Out1 : Outport
  wires:
  Sum3/1 -> Gain1/1
  Gain1/1 -> Discrete-Time Integrator/1
  Gain2/1 -> Sum3/2
  In1/1 -> Sum3/1
  Discrete-Time Integrator/1 -> Gain2/1, Out1/1

== system GFMUPS100k_CPP/Subsystem8 ==
  In1 : Inport
  Discrete-Time Integrator : DiscreteIntegrator  SampleTime=1/20000  ICPrevOutput=DiscIntNeverNeededParam  ICPrevScaledInput=DiscIntNeverNeededParam
  Gain1 : Gain  Gain=2*pi*50
  Gain2 : Gain
  Sum3 : Sum  Inputs=|+-
  Out1 : Outport
  wires:
  Discrete-Time Integrator/1 -> Out1/1, Gain2/1
  In1/1 -> Sum3/1
  Gain2/1 -> Sum3/2
  Gain1/1 -> Discrete-Time Integrator/1
  Sum3/1 -> Gain1/1

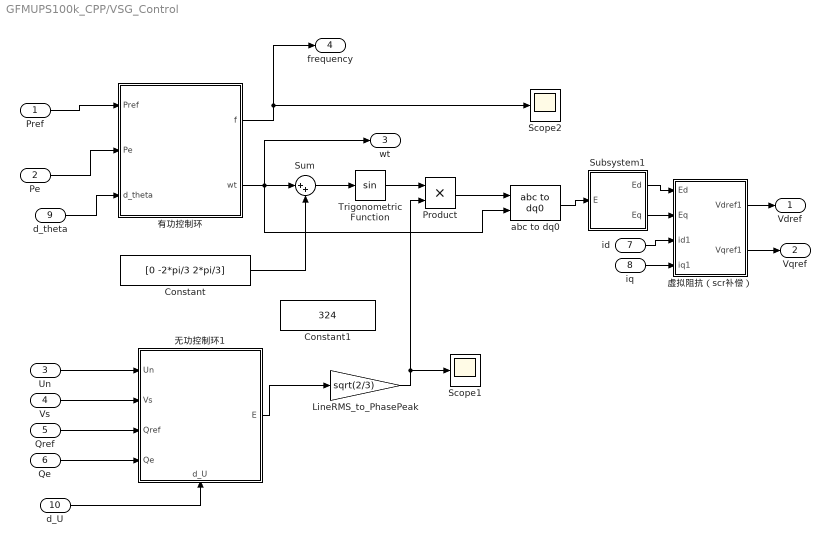
== system GFMUPS100k_CPP/VSG_Control ==
  Pref : Inport
  Pe : Inport  Port=2
  Un : Inport  Port=3
  Vs : Inport  Port=4
  Qref : Inport  Port=5
  Qe : Inport  Port=6
  id : Inport  Port=7
  iq : Inport  Port=8
  d_theta : Inport  Port=9
  d_U : Inport  Port=10
  Constant : Constant  Value=[0 -2*pi/3 2*pi/3]
  Constant1 : Constant  Value=324
  LineRMS_to_PhasePeak : Gain  Gain=sqrt(2/3)
  Product : Product
  Scope1 : Scope
  Scope2 : Scope
  Subsystem1 : Subsystem
  Sum : Sum  Inputs=|++
  Trigonometric Function : Trigonometry
  abc to dq0 : spsabctodq0Lib/abc to dq0  Alignment=90 degrees behind phase A axis
  无功控制环1 : Subsystem
      settings: PortSchema="{\"entries\":[{\"content\":{\"sides\":[{\"content\":{\"connectorIds\":[\"In1\",\"In2\",\"In3\",\"In4\"]},\"type\":\"ConnectorPlacement.EquallySpacedRectSide\",\"uuid\":\"5d331db0-156f-4c79-b59c-2964eff8acba\"},{\"content\":{\"connectorIds\":[\"Out1\"],\"side\":\"RIGHT\"},\"type\":\"ConnectorPlacement.EquallySpacedRectSide\",\"uuid\":\"187b12f5-effd-47ec-bb26-078b168957e5\"},{\"content\":{\"side\":\"TOP\"},\"type\":\"ConnectorPlacement.EquallySpacedRectSide\",\"uuid\":\"330c47bc-284a-4178-a4f6-6e435e4a7149\"},{\"content\":{\"connectorIds\":[\"In5\"],\"side\":\"BOTTOM\"},\"type\":\"ConnectorPlacement.EquallySpacedRectSide\",\"uuid\":\"0e044df9-336b-4f67-9480-ea34e9e33b74\"}]},\"type\":\"ConnectorPlacement.EquallySpacedConnector\",\"uuid\":\"e6089e41-3d81-472d-b808-d9560655865e\"}],\"packageUris\":[\"http://schema.mathworks.com/mf0/Connector/R2020b\"],\"version\":\"1.0\"}"
  有功控制环 : Subsystem
  虚拟阻抗（scr补偿） : Subsystem
  Vdref : Outport
  Vqref : Outport  Port=2
  wt : Outport  Port=3
  frequency : Outport  Port=4
  wires:
  无功控制环1/1(E) -> LineRMS_to_PhasePeak/1
  abc to dq0/1 -> Subsystem1/1(E)
  Sum/1 -> Trigonometric Function/1
  Qref/1 -> 无功控制环1/3(Qref)
  Trigonometric Function/1 -> Product/1
  Qe/1 -> 无功控制环1/4(Qe)
  Vs/1 -> 无功控制环1/2(Vs)
  Constant/1 -> Sum/2
  有功控制环/2(wt) -> wt/1, Sum/1, abc to dq0/2
  Un/1 -> 无功控制环1/1(Un)
  Product/1 -> abc to dq0/1
  有功控制环/1(f) -> frequency/1, Scope2/1
  Pref/1 -> 有功控制环/1(Pref)
  Pe/1 -> 有功控制环/2(Pe)
  Subsystem1/1(Ed) -> 虚拟阻抗（scr补偿）/1(Ed)
  Subsystem1/2(Eq) -> 虚拟阻抗（scr补偿）/2(Eq)
  iq/1 -> 虚拟阻抗（scr补偿）/4(iq1)
  id/1 -> 虚拟阻抗（scr补偿）/3(id1)
  虚拟阻抗（scr补偿）/1(Vdref1) -> Vdref/1
  虚拟阻抗（scr补偿）/2(Vqref1) -> Vqref/1
  d_theta/1 -> 有功控制环/3(d_theta)
  d_U/1 -> 无功控制环1/5(d_U)
  LineRMS_to_PhasePeak/1 -> Product/2, Scope1/1

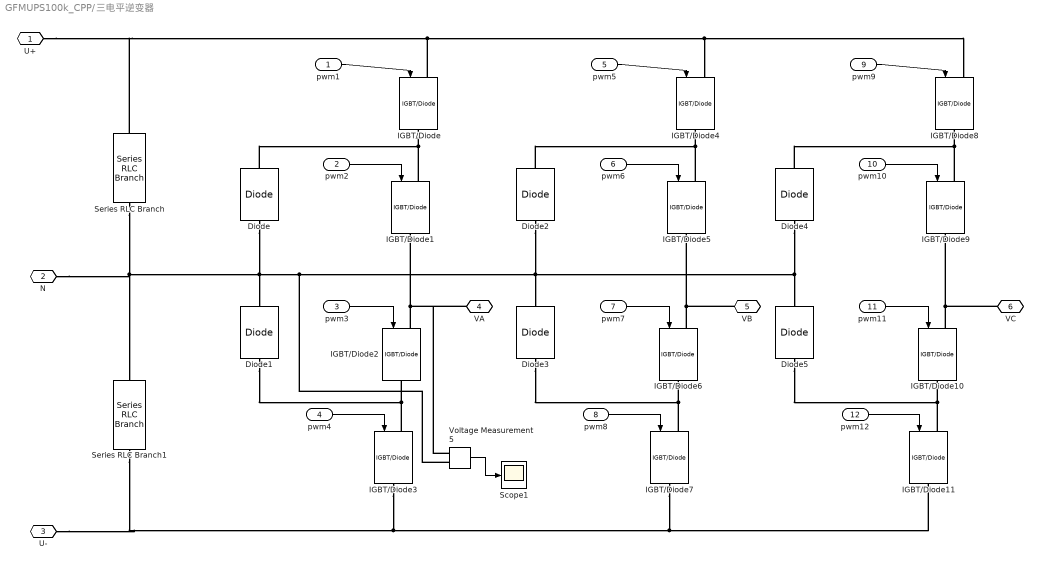
== system GFMUPS100k_CPP/三电平逆变器 ==
  pwm1 : Inport
  pwm2 : Inport  Port=2
  pwm3 : Inport  Port=3
  pwm4 : Inport  Port=4
  pwm5 : Inport  Port=5
  pwm6 : Inport  Port=6
  pwm7 : Inport  Port=7
  pwm8 : Inport  Port=8
  pwm9 : Inport  Port=9
  pwm10 : Inport  Port=10
  pwm11 : Inport  Port=11
  pwm12 : Inport  Port=12
  Diode{,1..5} (6 alike) : spsDiodeLib/Diode  Ron=0.001  Lon=0  Vf=0.8  IC=0  UseSnubber=0  Rs=500  Cs=250e-9  Measurements=off
  IGBT/Diode{,1..11} (12 alike) : spsIGBTDiodeLib/IGBT//Diode  Ron=1e-3  Rs=1e5  Cs=inf  Measurements=off
  Scope1 : Scope
  Series RLC Branch : spsSeriesRLCBranchLib/Series RLC Branch  LConnTagsString=__new0  RConnTagsString=__new0  BranchType=RC  Resistance=1e-3  Inductance=1e-3  SetiL0=off  InitialCurrent=0  Capacitance=4360e-6  Setx0=off  InitialVoltage=0  Measurements=None
  Series RLC Branch1 : spsSeriesRLCBranchLib/Series RLC Branch  LConnTagsString=__new0  RConnTagsString=__new0  BranchType=RC  Resistance=1e-3  Inductance=1e-3  SetiL0=off  InitialCurrent=0  Capacitance=4360e-6  Setx0=off  InitialVoltage=0  Measurements=None
  Voltage Measurement5 : spsVoltageMeasurementLib/Voltage Measurement  PhasorSimulation=off  OutputType=Complex  PSBequivalent=0
  U+ : PMIOPort  Side=Left
  N : PMIOPort  Port=2  Side=Left
  U- : PMIOPort  Port=3  Side=Left
  VA : PMIOPort  Port=4  Side=Right
  VB : PMIOPort  Port=5  Side=Right
  VC : PMIOPort  Port=6  Side=Right
  wires:
  pwm6/1 -> IGBT/Diode5/1
  pwm11/1 -> IGBT/Diode10/1
  pwm7/1 -> IGBT/Diode6/1
  pwm12/1 -> IGBT/Diode11/1
  pwm5/1 -> IGBT/Diode4/1
  pwm8/1 -> IGBT/Diode7/1
  pwm3/1 -> IGBT/Diode2/1
  pwm10/1 -> IGBT/Diode9/1
  pwm2/1 -> IGBT/Diode1/1
  pwm9/1 -> IGBT/Diode8/1
  Voltage Measurement5/1 -> Scope1/1
  pwm4/1 -> IGBT/Diode3/1
  pwm1/1 -> IGBT/Diode/1
  connections:
  Series RLC Branch/RConn1 -- N/RConn1 -- Series RLC Branch1/LConn1 -- Diode/LConn1 -- Voltage Measurement5/LConn2 -- Diode2/LConn1 -- Diode4/LConn1 -- Diode5/RConn1 -- Diode3/RConn1 -- Diode1/RConn1
  IGBT/Diode10/LConn1 -- VC/RConn1 -- IGBT/Diode9/RConn1
  Diode3/LConn1 -- IGBT/Diode7/LConn1 -- IGBT/Diode6/RConn1
  IGBT/Diode6/LConn1 -- VB/RConn1 -- IGBT/Diode5/RConn1
  IGBT/Diode1/LConn1 -- Diode/RConn1 -- IGBT/Diode/RConn1
  IGBT/Diode11/LConn1 -- Diode5/LConn1 -- IGBT/Diode10/RConn1
  IGBT/Diode3/RConn1 -- Series RLC Branch1/RConn1 -- U-/RConn1 -- IGBT/Diode7/RConn1 -- IGBT/Diode11/RConn1
  IGBT/Diode9/LConn1 -- Diode4/RConn1 -- IGBT/Diode8/RConn1
  IGBT/Diode2/LConn1 -- VA/RConn1 -- Voltage Measurement5/LConn1 -- IGBT/Diode1/RConn1
  Diode2/RConn1 -- IGBT/Diode5/LConn1 -- IGBT/Diode4/RConn1
  IGBT/Diode3/LConn1 -- Diode1/LConn1 -- IGBT/Diode2/RConn1
  IGBT/Diode/LConn1 -- Series RLC Branch/LConn1 -- U+/RConn1 -- IGBT/Diode8/LConn1 -- IGBT/Diode4/LConn1
